simulink model "test_SimulinkMdl3LPV_MPC"  (R2019b)
settings: Solver=FixedStepAuto  StartTime=0.0  StopTime=400  FixedStep=DT  RelTol=1e-3
values from neighbouring files (symbols this model uses):
  Cq = 0.0 0.0 0.0 0.0 0.0 0.0 0.0 0.0 0.0 0.0 0.0 0.0 0.0 0.0 0.0 0.0 0.0 0.0 0.0 0.0 0.0 0.0 0.0 0.0 0.0 0.0 0.0 0.0 0.0 0.0 0.0 0.0 0.0 0.0 0.0 0.0 0.0 0.0 0.0 0.0 0.0 0.0 0.0 0.0 0.0 0.0 0.0 0.0 0.0 0.0 0.0 0.0 0.0 0.0 0.0 0.0 0.0 0.0 0.0 0.0 0.0 0.0 0.0 0.0 0.0 0.0 0.0 0.0 0.0 0.0 0.0 0.0 0.0 0.0 0.0 0.0 0.0 0.0 0.0 0.0 0.0 0.0 0.0 0.0 0.0 0.0 0.0 0.0 0.0 0.0 0.0 0.0 0.0 0.0 0.0 0.0 0.0 0.0 0.0 0.0    [DD_test.sldd]    (also in testOutList.m = saveVarsMat.Cq)
  Drivetrain = struct    [dataDLR.m]
  DT = 0.008    [dataDLR.m]    (also in generateReport.m; initLPVParam.m; initWorkspace.m; runCalculateEvalCriteria.m)
  Lin_points : value not decoded    [DD_test.sldd]
  mu_old = zeros(2*N*nu,1)    [testCtrl.m]
  Ng = 97    [dataDLR.m]    (also in testCtrl.m)
  OutList = OutTable.Properties.VariableNames    [initLPVParam.m]    (also in testCtrl.m; testOutList.m = cell(40, 1); testqLPV.m = cell(40, 1))
  U = zeros(2*N,1)    [testCtrl.m]
  Xk07 = kron(ones(N,1),xk07)    [testCtrl.m]
  xk07 = [r7(1), r7(2), zeros(1,5),0]'    [testCtrl.m]
undefined symbols (not defined in the file or in its folder): Rotor_Lambda, Rotor_Lamda, Rotor_Pitch, strmatch
libraries: MdlLib_ProcessOutput x1
settings Model: ExtModeTrigMode=oneshot  ExtModeArmWhenConnect=off  Creator=Hazim Namik  LastModifiedBy=ditt_aj
settings DataIOCC: LimitDataPoints=on  SaveFormat=Array  ReturnWorkspaceOutputs=off
settings OptimizationCC: BlockReduction=off  BooleanDataType=off  LifeSpan=inf
settings DebuggingCC: SaveWithParameterizedLinksMsg=none  UnderspecifiedInitializationDetection=Classic  MergeDetectMultiDrivingBlocksExec=none  SignalResolutionControl=TryResolveAllWithWarning  SFUnexpectedBacktrackingDiag=warning  SFNoUnconditionalDefaultTransitionDiag=warning  SFExecutionAtInitializationDiag=none  ArithmeticOperatorsInVariantConditions=warning
settings HardwareCC: ProdBitPerPointer=32  ProdBitPerSizeT=32  ProdBitPerPtrDiffT=32  ProdLargestAtomicFloat=None  ProdIntDivRoundTo=Undefined  ProdEndianess=Unspecified  ProdWordSize=32  ProdHWDeviceType=32-bit Generic  TargetUnknown=on
settings ModelReferenceCC: PropagateSignalLabelsOutOfModel=off
settings SFSimCC: SimUseLocalCustomCode=off  CustomCodeUndefinedFunction=UseInterfaceOnly
settings RTWCC: RTWUseLocalCustomCode=off
settings CodeAppCC: StateflowObjectComments=on
settings GRTTargetCC: TargetLangStandard=C89/C90 (ANSI)  GeneratePreprocessorConditionals=Disable all
settings ConfigComp: CovMetricSettings=dw  CovHtmlReporting=on  CovSaveCumulativeToWorkspaceVar=on  CovSaveSingleToWorkspaceVar=on  CovExternalEMLEnable=off

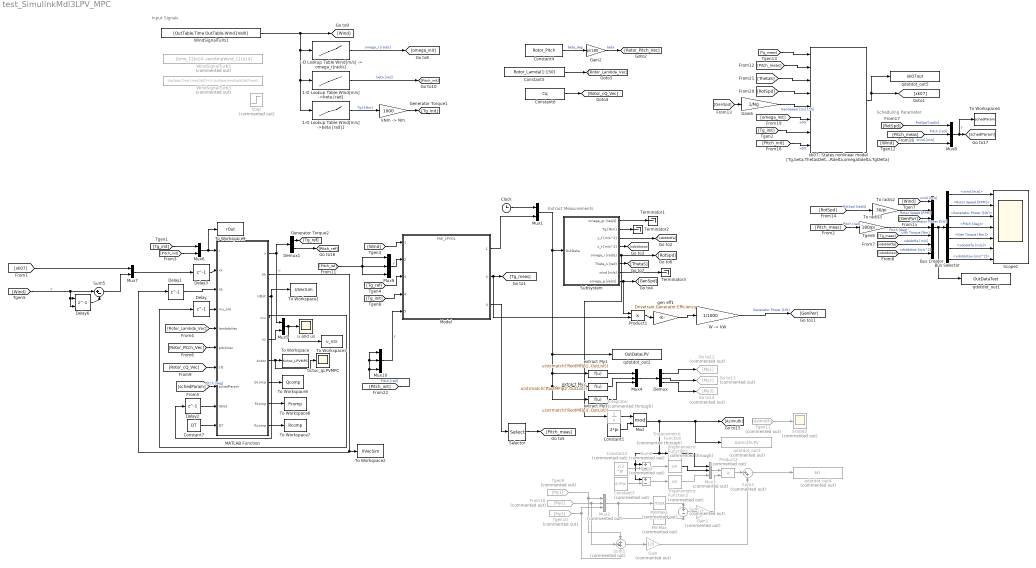
== system test_SimulinkMdl3LPV_MPC ==
  note: Extract Measurements
  note: Input Signals
  note: Scheduling Parameter
  "1-D Lookup Table Wind[m/s] -> omega_r[rad/s]" : Lookup_n-D  NumberOfTableDimensions=1  BreakpointsForDimension1=Lin_points.V  BreakpointsForDimension2=Rotor_Lambda  Table=Lin_points.RSpeed  InternalRulePriority=Speed  RndMeth=Simplest  InputSameDT=on
  1-D Lookup Table Wind[m/s] ->beta [rad] : Lookup_n-D  NumberOfTableDimensions=1  BreakpointsForDimension1=Lin_points.V  BreakpointsForDimension2=Rotor_Lambda  Table=Lin_points.Pitch  InternalRulePriority=Speed  RndMeth=Simplest  InputSameDT=on
  1-D Lookup Table Wind[m/s] ->beta [rad]1 : Lookup_n-D  NumberOfTableDimensions=1  BreakpointsForDimension1=Lin_points.V  BreakpointsForDimension2=Rotor_Lambda  Table=Lin_points.Torque  InternalRulePriority=Speed  RndMeth=Simplest  InputSameDT=on
  Bus Creator : BusCreator  Inputs=7
  Bus Selector : BusSelector  OutputSignals=wind [m/s],Rotor Speed [RPM],Generator Power [kW],Pitch [deg],Gen Torque [Nm],xdodotfa [m/s],xdotdotsw [m/s^2]
  Clock : Clock
  Constant1 : Constant  Value=2*pi
  Constant2 : Constant  Commented=on  Value=2/3 *pi
  Constant3 : Constant  Commented=on  Value=4/3*pi
  Constant4 : Constant  Value=Rotor_Pitch
  Constant5 : Constant  Value=Rotor_Lamda(1:150)
  Constant6 : Constant  Value=Cq
  Constant7 : Constant  Value=DT
  Delay : Delay  DelayLength=1  InitialCondition=mu_old
  Delay1 : Delay  DelayLength=1  InitialCondition=Xk07
  Delay2 : Delay  DelayLength=1  InitialCondition=U
  Delay3 : Delay  DelayLength=1  InitialCondition=xk07
  Delay6 : Delay  DelayLength=1  InitialConditionSource=Input port  InitialCondition=[0, Lin_points.Torque(1)]
      settings: InputPortMap=u0,p4
  Demux : Demux  Outputs=3
  Demux1 : Demux  Outputs=2
  From10 : From  Commented=on  GotoTag=My2
      settings: CloseFcn=tagdialog Close
  Gain : Gain  Commented=on  Gain=1/3
  Gain1 : Gain  Commented=on  Gain=1/2
  Gain2 : Gain  Gain=pi/180
  Gain6 : Gain  Gain=1/Ng
  Go to12 : Goto  Commented=on  GotoTag=My1
  Go to13 : Goto  Commented=on  GotoTag=My2
  Go to14 : Goto  Commented=on  GotoTag=My3
  Integrator : Integrator  Commented=through
  MATLAB Function : MATLAB Function  TreatAsAtomicUnit=on
  MinMax : MinMax  Commented=on
  MinMax1 : MinMax  Commented=on  Function=max
  Mod : Math  Operator=mod  SaturateOnIntegerOverflow=on
  Model : ModelReference  ModelNameDialog=Mdl_LPVOL.slx  SimulationMode=Normal  ModelReferenceVersion=1.38
  Mux{1,5..7} (4 alike) : Mux  Inputs=2
  Mux{4,8..10} (4 alike) : Mux  Inputs=3
  Mux2 : Mux  Commented=on  Inputs=3
  Mux3 : Mux  Commented=on  Inputs=3
  Product1 : Product  RndMeth=Zero
  Product2 : Product  Commented=on  RndMeth=Zero
  Scope1 : Scope  NumInputPorts=7
      settings: Tag=Scope
  Scope3 : Scope  Commented=on
  Selector : Selector  InputPortWidth=3  IndexOptions=Index vector (dialog)  Indices=1  OutputSizes=1
  Step : Step  Commented=on  Time=5  Before=11  After=12  SampleTime=0
  Subsystem : Subsystem
  Sum : Sum  Commented=on  Inputs=+-
  Sum1 : Sum  Commented=on  Inputs=+++
  Sum2 : Sum  Commented=on  Inputs=+-
  Sum3 : Sum  Commented=on  Inputs=+-
  Sum4 : Sum  Commented=on  Inputs=|++
  Sum5 : Sum  Inputs=|+-
  Terminator1 : Terminator
  Terminator2 : Terminator
  Terminator3 : Terminator
  Tgen10 : From  Commented=on  GotoTag=My3
      settings: CloseFcn=tagdialog Close
  Tgen11 : From  Commented=on  GotoTag=Azimuth
      settings: CloseFcn=tagdialog Close
  Tgen9 : From  Commented=on  GotoTag=My1
      settings: CloseFcn=tagdialog Close
  To Workspace : ToWorkspace  VariableName=tictoc_LPVMPC  SaveFormat=Timeseries  SampleTime=-1
  To Workspace1 : ToWorkspace  VariableName=UVecSim  SampleTime=-1
  To Workspace2 : ToWorkspace  VariableName=XVecSim  SampleTime=-1
  To Workspace3 : ToWorkspace  VariableName=u_uss  SampleTime=-1
      settings: Save2DSignal=2-D array (concatenate along first dimension)
  To Workspace4 : ToWorkspace  VariableName=schedParam  SampleTime=-1
      settings: Save2DSignal=2-D array (concatenate along first dimension)
  To Workspace5 : ToWorkspace  VariableName=Qcomp  SampleTime=-1
      settings: Save2DSignal=2-D array (concatenate along first dimension)
  To Workspace6 : ToWorkspace  VariableName=Pcomp  SampleTime=-1
      settings: Save2DSignal=2-D array (concatenate along first dimension)
  To Workspace7 : ToWorkspace  VariableName=Rcomp  SampleTime=-1
      settings: Save2DSignal=2-D array (concatenate along first dimension)
  To Workspace9 : ToWorkspace  VariableName=rOut  SampleTime=-1
  To rad/s2 : Gain  Gain=30/pi
  To rad/s3 : Gain  Gain=180/pi
  Trigonometric Function : Trigonometry  Commented=through
  Trigonometric Function1 : Trigonometry  Commented=through
  Trigonometric Function2 : Trigonometry  Commented=on
  "W -> kW" : Gain  Gain=1/1000
  WindSignalTurb1 : FromWorkspace  VariableName=[OutTable.Time OutTable.Wind1VelX]  SampleTime=DT  OutputAfterFinalValue=Holding final value
  WindSignalTurb2 : FromWorkspace  Commented=on  VariableName=[time_11to14' vectAmpWind_11to14]  SampleTime=DT  OutputAfterFinalValue=Holding final value
  WindSignalTurb3 : FromWorkspace  Commented=on  VariableName=[OutTable.Time(1:(end-20/DT+1)),OutTable.Wind1VelX(20/DT:end)]  SampleTime=DT  OutputAfterFinalValue=Holding final value
  extract My1 : Fcn  Expr=u(strmatch('RootMFlp1',OutList))
  extract My2 : Fcn  Expr=u(strmatch('RootMFlp2',OutList))
  extract My3 : Fcn  Expr=u(strmatch('RootMFlp3',OutList))
  gen eff1 : Gain  Gain=Drivetrain.Generator.Efficiency
  "kNm -> Nm" : Gain  Gain=1000
  qdotdot_out1 : ToWorkspace  VariableName=OutDataTest  SampleTime=-1
  qdotdot_out2 : ToWorkspace  VariableName=OutDataLPV  SampleTime=-1
  qdotdot_out3 : ToWorkspace  Commented=on  VariableName=AzimuthLPV  SampleTime=-1
  qdotdot_out4 : ToWorkspace  Commented=on  VariableName=MY  SampleTime=-1
  qdotdot_out5 : ToWorkspace  VariableName=xk07out  SampleTime=-1
  tictoc_qLPVMPC : Scope
  u and us : Scope
  xk07: States nonlinear model [Tg,beta,ThetasDelta,omegaRdelta,omegaGdelta,TgDelta] : MdlLib_ProcessOutput/xk07: States nonlinear model [Tg,beta,ThetasDelta,omegaRdelta,omegaGdelta,TgDelta]  SystemSampleTime=-1  Latency=0  AutoFrameSizeCalculation=off
  wires:
  "1-D Lookup Table Wind[m/s] -> omega_r[rad/s]"/1 -> [omega_init]  "omega_r [rad/s]"
  1-D Lookup Table Wind[m/s] ->beta [rad]1/1 -> "kNm -> Nm"/1  "Tg [kNm]"
  WindSignalTurb1/1 -> [Wind], "1-D Lookup Table Wind[m/s] -> omega_r[rad/s]"/1, 1-D Lookup Table Wind[m/s] ->beta [rad]/1, 1-D Lookup Table Wind[m/s] ->beta [rad]1/1
  "kNm -> Nm"/1 -> [Tg_init]
  1-D Lookup Table Wind[m/s] ->beta [rad]/1 -> [Pitch_init]  "beta [rad]"
  [Tg_init] -> Model/4
  [Wind] -> Model/1
  Subsystem/1(omega_gr [rad/s]) -> Terminator1/1
  Subsystem/8(omega_g [rad/s]) -> [GenSpd], Product1/1
  Subsystem/3(y_t [m/s^2]) -> [xdotdotfa]
  Subsystem/6(Theta_s [rad]) -> [ThetaS]
  Model/3 -> Selector/1
  [Tg_ref] -> Model/3
  Bus Selector/3 -> Scope1/3  "<Generator Power [kW]>"
  Bus Selector/7 -> Scope1/7  "<xdotdotsw [m/s^2]>"
  To rad/s2/1 -> Bus Creator/2  "Rotor Speed [RPM]"
  [GenPwr] -> Bus Creator/3  "Generator Power [kW]"
  [Tg_meas] -> Bus Creator/5  "Gen Torque [Nm]"
  [xdotdotsw] -> Bus Creator/7  "xdotdotsw [m/s^2]"
  Bus Creator/1 -> Bus Selector/1, qdotdot_out1/1
  Bus Selector/6 -> Scope1/6  "<xdodotfa [m/s]>"
  To rad/s3/1 -> Bus Creator/4  "Pitch [deg]"
  [Wind] -> Bus Creator/1  "wind [m/s]"
  Bus Selector/4 -> Scope1/4  "<Pitch [deg]>"
  [Pitch_meas] -> To rad/s3/1  "Pitch [rad]"
  [xdotdotfa] -> Bus Creator/6  "xdodotfa [m/s]"
  [RotSpd] -> To rad/s2/1  "RotSpd [rad/s]"
  Bus Selector/2 -> Scope1/2  "<Rotor Speed [RPM]>"
  Bus Selector/5 -> Scope1/5  "<Gen Torque [Nm]>"
  Bus Selector/1 -> Scope1/1  "<wind [m/s]>"
  Mux1/1 -> extract My3/1, extract My2/1, extract My1/1, qdotdot_out2/1, Subsystem/1(OutData)
  Clock/1 -> Mux1/1
  Model/1 -> Mux1/2
  "W -> kW"/1 -> [GenPwr]  "Generator Power [kW]"
  gen eff1/1 -> "W -> kW"/1
  Product1/1 -> gen eff1/1
  Model/2 -> Product1/2, [Tg_meas]
  Subsystem/2(Tg [N/m]) -> Terminator2/1
  Subsystem/4(x_t [m/s^2]) -> [xdotdotsw]
  Subsystem/7(wind [m/s]) -> Terminator3/1
  Tgen10/1 -> Sum1/3, Mux2/3
  Tgen9/1 -> Sum1/1, Mux2/1
  From10/1 -> Mux2/2, Sum1/2
  Mux2/1 -> MinMax1/1, MinMax/1
  Tgen11/1 -> Scope3/1
  Integrator/1 -> Mod/1
  Constant1/1 -> Mod/2
  Subsystem/5(omega_r [rad/s]) -> [RotSpd], Integrator/1
  Mod/1 -> Sum3/1, Sum2/1, Trigonometric Function/1, qdotdot_out3/1, [Azimuth]
  MinMax1/1 -> Sum/1
  MinMax/1 -> Sum/2
  Sum/1 -> Gain1/1
  Sum1/1 -> Gain/1
  Gain/1 -> Sum4/2
  Trigonometric Function/1 -> Mux3/1
  Constant2/1 -> Sum2/2
  Constant3/1 -> Sum3/2
  Sum2/1 -> Trigonometric Function1/1
  Sum3/1 -> Trigonometric Function2/1
  Gain1/1 -> Product2/2
  Trigonometric Function1/1 -> Mux3/2
  Trigonometric Function2/1 -> Mux3/3
  Mux3/1 -> Product2/1
  Product2/1 -> Sum4/1
  Sum4/1 -> qdotdot_out4/1
  extract My1/1 -> Mux4/1
  extract My2/1 -> Mux4/2
  extract My3/1 -> Mux4/3
  Demux/3 -> Go to14/1
  Demux/1 -> Go to12/1
  Demux/2 -> Go to13/1
  Mux4/1 -> Demux/1
  Constant5/1 -> [Rotor_Lambda_Vec]
  Constant4/1 -> Gain2/1  "beta_deg"
  Constant6/1 -> [Rotor_cQ_Vec]
  Gain2/1 -> [Rotor_Pitch_Vec]  "beta"
  [Rotor_Lambda_Vec] -> MATLAB Function/5(lambdaVec)
  [xk07] -> Mux7/1
  Delay/1 -> MATLAB Function/4(mu_old)
  MATLAB Function/2(Xk) -> Delay1/1, To Workspace2/1
  Mux5/1 -> u and us/1, To Workspace3/1
  Delay3/1 -> MATLAB Function/2(xk)
  Demux1/1 -> [Tg_ref]
  Delay6/1 -> Sum5/2
  MATLAB Function/8(Pcomp) -> To Workspace6/1
  [Pitch_init] -> Mux6/2
  [Tg_init] -> Mux6/1
  MATLAB Function/9(Rcomp) -> To Workspace7/1
  Mux7/1 -> Delay3/1
  Demux1/2 -> [Pitch_ref]
  Mux6/1 -> To Workspace9/1, MATLAB Function/1(r)
  [schedParam] -> MATLAB Function/8(schedParam)  "Pitch [deg]"
  [Rotor_cQ_Vec] -> MATLAB Function/7(cQ)
  Delay2/1 -> MATLAB Function/9("UDot ")
  Sum5/1 -> Mux7/2
  MATLAB Function/7(Qcomp) -> To Workspace5/1
  MATLAB Function/6(tictoc) -> tictoc_qLPVMPC/1, To Workspace/1
  [Wind] -> Delay6/2, Delay6/1, Sum5/1  "y"
  Delay1/1 -> MATLAB Function/3("Xk ")
  MATLAB Function/1(u) -> Demux1/1, Mux5/1  "u"
  Constant7/1 -> MATLAB Function/10(DT)
  MATLAB Function/4(mu) -> Delay/1
  [Rotor_Pitch_Vec] -> MATLAB Function/6(pitchVec)
  MATLAB Function/3(UDot) -> Delay2/1, To Workspace1/1
  MATLAB Function/5(us) -> Mux5/2
  Gain6/1 -> xk07: States nonlinear model [Tg,beta,ThetasDelta,omegaRdelta,omegaGdelta,TgDelta]/5  "GenSpeed [1/s] LSS]"
  Mux8/1 -> To Workspace4/1, [schedParam]  "y"
  [RotSpd] -> xk07: States nonlinear model [Tg,beta,ThetasDelta,omegaRdelta,omegaGdelta,TgDelta]/4
  [Wind] -> Mux8/3  "Wind [m/s]"
  [Pitch_meas] -> xk07: States nonlinear model [Tg,beta,ThetasDelta,omegaRdelta,omegaGdelta,TgDelta]/2
  [Tg_meas] -> xk07: States nonlinear model [Tg,beta,ThetasDelta,omegaRdelta,omegaGdelta,TgDelta]/1
  [RotSpd] -> Mux8/1  "RotSpd [rad/s]"
  [ThetaS] -> xk07: States nonlinear model [Tg,beta,ThetasDelta,omegaRdelta,omegaGdelta,TgDelta]/3
  [Pitch_init] -> xk07: States nonlinear model [Tg,beta,ThetasDelta,omegaRdelta,omegaGdelta,TgDelta]/8  "xdot"
  xk07: States nonlinear model [Tg,beta,ThetasDelta,omegaRdelta,omegaGdelta,TgDelta]/1 -> [xk07], qdotdot_out5/1
  [Pitch_meas] -> Mux8/2  "Pitch [rad]"
  [Tg_init] -> xk07: States nonlinear model [Tg,beta,ThetasDelta,omegaRdelta,omegaGdelta,TgDelta]/7
  [omega_init] -> xk07: States nonlinear model [Tg,beta,ThetasDelta,omegaRdelta,omegaGdelta,TgDelta]/6  "xdot"
  [GenSpd] -> Gain6/1
  Mux9/1 -> Model/2  "y"
  [Pitch_ref] -> Mux9/3, Mux9/2, Mux9/1
  Selector/1 -> [Pitch_meas]
  Mux10/1 -> Model/5  "y"
  [Pitch_init] -> Mux10/3, Mux10/1, Mux10/2  "Pitch [rad]"

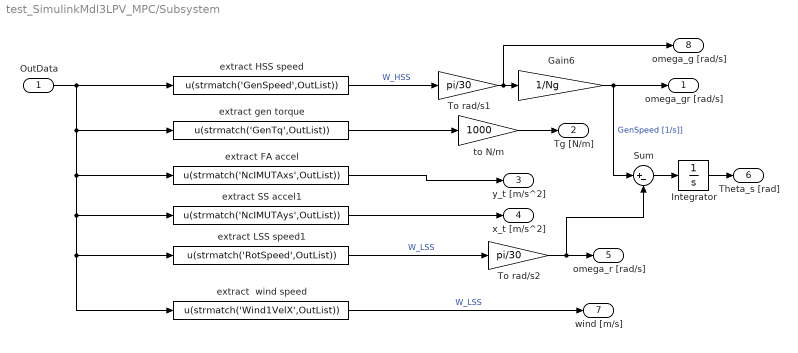
== system test_SimulinkMdl3LPV_MPC/Subsystem ==
  OutData : Inport
  Gain6 : Gain  Gain=1/Ng
  Integrator : Integrator
  Sum : Sum  Inputs=|+-
  To rad/s1 : Gain  Gain=pi/30
  To rad/s2 : Gain  Gain=pi/30
  extract  wind speed : Fcn  Expr=u(strmatch('Wind1VelX',OutList))
  extract FA accel : Fcn  Expr=u(strmatch('NcIMUTAxs',OutList))
  extract HSS speed : Fcn  Expr=u(strmatch('GenSpeed',OutList))
  extract LSS speed1 : Fcn  Expr=u(strmatch('RotSpeed',OutList))
  extract SS accel1 : Fcn  Expr=u(strmatch('NcIMUTAys',OutList))
  extract gen torque : Fcn  Expr=u(strmatch('GenTq',OutList))
  to N/m : Gain  Gain=1000
  omega_gr [rad/s] : Outport  VectorParamsAs1DForOutWhenUnconnected=off
  Tg [N/m] : Outport  Port=2  VectorParamsAs1DForOutWhenUnconnected=off
  y_t [m/s^2] : Outport  Port=3  VectorParamsAs1DForOutWhenUnconnected=off
  x_t [m/s^2] : Outport  Port=4  VectorParamsAs1DForOutWhenUnconnected=off
  omega_r [rad/s] : Outport  Port=5  VectorParamsAs1DForOutWhenUnconnected=off
  Theta_s [rad] : Outport  Port=6  VectorParamsAs1DForOutWhenUnconnected=off
  wind [m/s] : Outport  Port=7  VectorParamsAs1DForOutWhenUnconnected=off
  omega_g [rad/s] : Outport  Port=8  VectorParamsAs1DForOutWhenUnconnected=off
  wires:
  to N/m/1 -> Tg [N/m]/1
  OutData/1 -> extract HSS speed/1, extract gen torque/1, extract  wind speed/1, extract LSS speed1/1, extract SS accel1/1, extract FA accel/1
  extract FA accel/1 -> y_t [m/s^2]/1
  extract HSS speed/1 -> To rad/s1/1  "W_HSS"
  extract gen torque/1 -> to N/m/1
  extract SS accel1/1 -> x_t [m/s^2]/1
  To rad/s1/1 -> omega_g [rad/s]/1, Gain6/1
  extract LSS speed1/1 -> To rad/s2/1  "W_LSS"
  Gain6/1 -> omega_gr [rad/s]/1, Sum/1  "GenSpeed [1/s]]"
  To rad/s2/1 -> Sum/2, omega_r [rad/s]/1
  Sum/1 -> Integrator/1
  Integrator/1 -> Theta_s [rad]/1
  extract  wind speed/1 -> wind [m/s]/1  "W_LSS"

== matlab function test_SimulinkMdl3LPV_MPC/MATLAB Function ==
  settings: updateMethod=DISCRETE
  data: r input; u output; xk input; Xk input; mu_old input; lambdaVec input; pitchVec input; cQ input; schedParam input; UDot input; DT input; Xk output; UDot output; mu output; us output; tictoc output; Qcomp output; Pcomp output; Rcomp output
function [u,Xk,UDot,mu,us,tictoc, Qcomp,Pcomp,Rcomp]= qLPVMPC_WECS_beta(r,xk,Xk,mu_old,lambdaVec,pitchVec,cQ,schedParam,UDot,DT)
% MATLAB_Function calculates controller output u. It turns the QP into a 
% linear complementarity problem (LCP) and solves it with Lemke's algorithm.
%
% Inputs: * r: reference
%         * xk: quasiLPV KF state estimates
%         * Xk: Xko(= L*xk+S*U) delayed by one sample timestep
%         * mu_old: mu delayed by one sample timestep
%         * lambdaVec: lambda vector for cQ LUT 
%         * pitchVec: pitch vector for cQ LUT 
%         * cQ: torque coefficients LUT matrix
%         * schedParam: current values [omegaR, beta, V]
%         * U: U (from Xko = L*xk+S*U) delayed by one sample timestep
%
% Outputs: * u: controller output at current time step
%          * Xko: Future state trajectory (L*xk+S*U)
%          * U: Future input trajectory 
%          * mu: Result Lemke's algorithm/LCP: M mu +q >=0, mu>=0, mu'(Mmu+q)=0
%          * us: xuss(end) from xuss = [eye(4)-Ass -Bss;[1 0 0 0] 0]\[Bss*d;1]
%          * tictoc: tic-toc result

% Pablo S.G. Cisneros, Herbert Werner, ICS TUHH

%#codegen
coder.extrinsic('tic');
coder.extrinsic('toc');
tictoc = 0;
tic

%% Init N, Q, R
N = 40;
q_ = [1 10^4 0 10^3 10^3 0 0 0]; %[10^4 0.1 1 1 100 0.1 0]; %q_ = [100 1000 1 0.01 0]; 7.351e+02 1.000e+00 1.938e+09 1.625e+08 1.491e+08 1.657e+03
r_ = [1 10^4]; %[10^7,0.1];
R_ = kron(eye(N),diag(r_)); %R_ = 1000*eye(N); 
p = 10^3*q_; %P = 1000*diag(q_);

Ulim = repmat([20000,8 * pi/180]',2*N,1); %rate constraints 

Control_Pitch_Max = 90 /180 * pi;
Control_Pitch_Min = 0 /180 * pi;
Control_Torque_Limit = 47403;
Control_Torque_Min = 200;

% isBetaState = 0;
% nx = 4 + isBetaState; % number states plant: ThetaS,omegaR,omegaG,Tg
% ny = 2 + isBetaState; % number of outputs plant omegaG,Tg
nxA = 8;% nx + ny +clc 1; %number states augmented plant 
nu = 2; % plant inputs: Tg_ref, beta_ref

%% Shift Xk
Xk(1:end-nxA) = Xk(nxA+1:end); 
UDot(1:end-nu) = UDot(nu+1:end);
%Xk(1:nxA)

%% Calculate input u_dot_s = 0  and steady state x = r
us = [0;0]; %xuss(nxA+1:nxA+2); % xuss = [eye(size(Ass))-Ass -Bss;[1 0 0 0] 0] \ [Bss*d;reference];

iterations = 1; % omega_ref(Vest), Tg_ref(Vest)
refVec = zeros(nxA,1);
refVec(1:2) = r;
ref = repmat(refVec,N,1); %ref = kron(ones(N,1),[r; 0; 0; 0;0]);

for i = 1:iterations
    [L,S,H,g] = HSqLd_WT_beta(N,q_,R_,p,xk,Xk,DT,ref,us,lambdaVec,pitchVec,cQ,schedParam,UDot);
    
    %% %%%%%%Turn QP into LCP and solve it%%%%%%%%%
    Ac_ = [-eye(N*nu);eye(N*nu)];
    bc_ = - Ulim;
    Hi = eye(size(H,1))/H;
    M = Ac_*Hi*Ac_';
    q = -Ac_*Hi*g - bc_;
 
    mu = lemke(M,q,mu_old);
 
    UDot = Hi*(Ac_'*mu-g);
    UDot(isnan(UDot)) = 0;
    
    %% %%%%%%%%%%%%%%%%%%%%%%%%%%%%%%%%%%%%%%%%%%%%    
    Xk = L*xk+S*UDot;
end

u =  [ min(max(UDot(1) + Xk(1), Control_Torque_Min),Control_Torque_Limit),... % torque
min( max(UDot(2) + Xk(2), Control_Pitch_Min),Control_Pitch_Max)]'; % pitch

tictoc = toc;

% For debugging
%%%%%%%%%%% Compute Hessian H, derivative g = dJk/dUk %%
% min Jk(Uk) s.t. h1(Uk) = 0, h2(Uk) < 0, at current estimate xl
% <=> min( x'H(xl)x + g(xl)x s.t. dh1(xl)x+h1(xl)=0, dh2(xl)x+h2(xl)< 0
% with 
% Jk = (Lx+SUk-Xss)'Q(Lx+SUk-Xss) +(Uk-Uss)'R(Uk-Uss) + Psi
% dJk/dUk = 2S'Q (Lx+SUk-Xss) + 2R(Uk-Uss) 
diffX = Xk(1:(end - nxA)) - ref(1:(end -nxA));
diffXEnd = Xk((end - nxA +1):end) - ref((end - nxA +1):end);

% Q_ = kron(eye(N-1),diag(q_));
% Qcomp = diffX' * Q_ * diffX;
% Pcomp = diffXEnd' * diag(p)* diffXEnd;
% Rcomp = U' * R_ * U;

diffXMat = sum(reshape(diffX.^2, nxA, N-1),2);
UMat = sum(reshape(UDot.^2, 2, N),2);

Qcomp = diffXMat' .* q_;
Pcomp = (diffXEnd') .^2  .* p;
Rcomp = UMat' .* r_;
